simulink model "sm_car_"  (R2026b)
settings: Solver=ode23t  StopTime=100  MaxStep=0.4  AbsTol=1e-3  EnableMultiTasking=on
PreLoadFcn:
  | % Due to usability issue in Repeating Sequence block
  | warning('off','Simulink:Masking:Invalid');
  | 
  | % Eliminate unnecessary warnings in inactive variants
  | % Warnings generated only if you click through inactive variant
  | warning('off','MATLAB:nonExistentField');
  | warning('off','Simulink:Parameters:BlkParamUndefined');
PostLoadFcn:
  | set_param([bdroot '/Vehicle'],'popup_trailer','Off')
  | warning('off','sm:sli:setup:compile:LocalSolverNotSupported')
  | %sm_car_config_maneuver(bdroot,'WOT Braking');
  | sm_car_config_vehicle(bdroot,'false');
  | sm_car_config_logging(bdroot);
InitFcn:
  | sm_car_config_camera;
  | Vehicle = sm_car_vehcfg_checkConfig(Vehicle);
  | sm_car_check_tire_model(bdroot);
StartFcn:
  | tic;
StopFcn:
  | Elapsed_Sim_Time = toc;
  | % disp(['Elapsed Sim Time = ' num2str(Elapsed_Sim_Time)]);
undefined symbols (not defined in the file or in its folder): acc_theta, accel_ramp_rate, Axle1D, AxleIn, Camera, Control, Driver, Init, Maneuver, Pedal, Scene, ShaftL1, ShaftL2, ShaftR1, ShaftR2, Visual, X, xy_data_car_side, Y, Z
libraries: sm_lib x290, fl_lib x171, nesl_utility x144, simulink x60, simulink_extras x14, sdl_lib x14, SimscapeFluids_lib x7, Damper_Element x4, Tire_1x2x x4, ee_lib x3, Scene_Utilities x3, sharedTrackingLibrary x2
(part 20 of 22)

== system sm_car_/Vehicle/Vehicle/Chassis/Spring/Decoupled/Spring A1 Roll/Linear ==
  note: Sensing
  Ctrl : Inport
  Displacement Spring : fl_lib/Mechanical/Mechanical Sensors/Ideal Translational Motion Sensor  reference=foundation.enum.MeasurementReference.difference  acceleration_port=false  velocity_port=true  position_port=true  offset=spr_len0 m
  Force Spring : fl_lib/Mechanical/Mechanical Sensors/Ideal Force Sensor
  PS Term Motion v : fl_lib/Physical Signals/Sinks/PS Terminator
  PS-Simulink Converter : nesl_utility/PS-Simulink Converter  PhysicalDomain=network_engine_domain  SubClassName=ps_output  LeftPortType=input  RightPortType=output  PseudoPeriodic=off  Frequencies=[]  VectorFormat=1-D array  Unit=m  AffineConversion=off
  PS-Simulink Converter1 : nesl_utility/PS-Simulink Converter  PhysicalDomain=network_engine_domain  SubClassName=ps_output  LeftPortType=input  RightPortType=output  PseudoPeriodic=off  Frequencies=[]  VectorFormat=1-D array  Unit=N  AffineConversion=off
  Spring : fl_lib/Mechanical/Translational Elements/Translational Spring  spr_rate=spr_k N/m  v_specify=off  v_priority=None  v=0 m/s  v_nominal_specify=off  v_nominal_value=1  v_nominal_unit=m/s  f_specify=off  f_priority=None  f=0 N  f_nominal_specify=off  f_nominal_value=1  f_nominal_unit=N  x_specify=on  x_priority=High  x=-spr_def0 m  x_nominal_specify=off  x_nominal_value=1  x_nominal_unit=m
  Terminator : Terminator
  R : PMIOPort  Side=Left
  C : PMIOPort  Port=2  Side=Right
  Out Bus Element : Outport  VectorParamsAs1DForOutWhenUnconnected=off  PortName=meas  Element=xSpring
  Out Bus Element1 : Outport  VectorParamsAs1DForOutWhenUnconnected=off  PortName=meas  Element=FSpring
  wires:
  PS-Simulink Converter1/1 -> Out Bus Element1/1
  Ctrl/1 -> Terminator/1
  PS-Simulink Converter/1 -> Out Bus Element/1
  connections:
  Spring/LConn1 -- R/RConn1 -- Displacement Spring/LConn1
  Spring/RConn1 -- Force Spring/RConn1 -- Displacement Spring/RConn1
  Force Spring/LConn1 -- C/RConn1
  PS-Simulink Converter1/LConn1 -- Force Spring/RConn2
  Displacement Spring/RConn2 -- PS Term Motion v/LConn1
  Displacement Spring/RConn3 -- PS-Simulink Converter/LConn1

== system sm_car_/Vehicle/Vehicle/Chassis/Spring/Decoupled/Spring A1 Roll/No Spring ==
  note: Sensor inserted simply to ensure
      | all blocks are connected to a network
  Ctrl : Inport
  Constant : Constant  Value=0
  Constant1 : Constant  Value=0
  Ideal Translational Motion Sensor : fl_lib/Mechanical/Mechanical Sensors/Ideal Translational Motion Sensor  reference=foundation.enum.MeasurementReference.difference  acceleration_port=false  velocity_port=true  position_port=true  offset=0 m
  PS-Simulink Converter : nesl_utility/PS-Simulink Converter  PhysicalDomain=network_engine_domain  SubClassName=ps_output  LeftPortType=input  RightPortType=output  PseudoPeriodic=off  Frequencies=[]  VectorFormat=1-D array  Unit=1  AffineConversion=off
  PS-Simulink Converter1 : nesl_utility/PS-Simulink Converter  PhysicalDomain=network_engine_domain  SubClassName=ps_output  LeftPortType=input  RightPortType=output  PseudoPeriodic=off  Frequencies=[]  VectorFormat=1-D array  Unit=1  AffineConversion=off
  Terminator : Terminator
  Terminator1 : Terminator
  Terminator2 : Terminator
  R : PMIOPort  Side=Left
  C : PMIOPort  Port=2  Side=Right
  Out Bus Element : Outport  VectorParamsAs1DForOutWhenUnconnected=off  PortName=meas  Element=xSpring
  Out Bus Element1 : Outport  VectorParamsAs1DForOutWhenUnconnected=off  PortName=meas  Element=FSpring
  wires:
  PS-Simulink Converter/1 -> Terminator1/1
  PS-Simulink Converter1/1 -> Terminator2/1
  Constant1/1 -> Out Bus Element/1
  Ctrl/1 -> Terminator/1
  Constant/1 -> Out Bus Element1/1
  connections:
  Ideal Translational Motion Sensor/RConn2 -- PS-Simulink Converter/LConn1
  PS-Simulink Converter1/LConn1 -- Ideal Translational Motion Sensor/RConn3
  C/RConn1 -- Ideal Translational Motion Sensor/RConn1
  R/RConn1 -- Ideal Translational Motion Sensor/LConn1

== system sm_car_/Vehicle/Vehicle/Chassis/Spring/Decoupled/Spring A1 Roll/Nonlinear ==
  note: Sensing
  Ctrl : Inport
  Displacement Spring : fl_lib/Mechanical/Mechanical Sensors/Ideal Translational Motion Sensor  reference=foundation.enum.MeasurementReference.difference  acceleration_port=false  velocity_port=true  position_port=true  offset=spr_len0 m
  Force Spring : fl_lib/Mechanical/Mechanical Sensors/Ideal Force Sensor
  PS Term Motion v : fl_lib/Physical Signals/Sinks/PS Terminator
  PS-Simulink Converter : nesl_utility/PS-Simulink Converter  PhysicalDomain=network_engine_domain  SubClassName=ps_output  LeftPortType=input  RightPortType=output  PseudoPeriodic=off  Frequencies=[]  VectorFormat=1-D array  Unit=m  AffineConversion=off
  PS-Simulink Converter1 : nesl_utility/PS-Simulink Converter  PhysicalDomain=network_engine_domain  SubClassName=ps_output  LeftPortType=input  RightPortType=output  PseudoPeriodic=off  Frequencies=[]  VectorFormat=1-D array  Unit=N  AffineConversion=off
  Spring : sdl_lib/Couplings & Drives/Springs & Dampers/Nonlinear Translational Spring  parameterization=2  symmetry=1  coefficient_vector=[100, 0, 10, 0, 1] N/m  tension_coefficient_vector=[100, 0, 10, 0, 1] N/m  compression_coefficient_vector=[1000, -10, 100, 0, 0] N/m  deformation_vector=deformation_vector m  force_vector=force_vector N  interp_method=simscape.enum.interpolation.linear  extrap_method=simscape.enum.extrapolation.linear  x_specify=on  x_priority=High  x=-spr_def0 m  x_nominal_specify=off  x_nominal_value=1  x_nominal_unit=m
  Terminator : Terminator
  R : PMIOPort  Side=Left
  C : PMIOPort  Port=2  Side=Right
  Out Bus Element : Outport  VectorParamsAs1DForOutWhenUnconnected=off  PortName=meas  Element=xSpring
  Out Bus Element1 : Outport  VectorParamsAs1DForOutWhenUnconnected=off  PortName=meas  Element=FSpring
  wires:
  PS-Simulink Converter/1 -> Out Bus Element/1
  Ctrl/1 -> Terminator/1
  PS-Simulink Converter1/1 -> Out Bus Element1/1
  connections:
  Displacement Spring/RConn3 -- PS-Simulink Converter/LConn1
  Displacement Spring/RConn2 -- PS Term Motion v/LConn1
  PS-Simulink Converter1/LConn1 -- Force Spring/RConn2
  Force Spring/LConn1 -- C/RConn1
  Displacement Spring/RConn1 -- Force Spring/RConn1 -- Spring/RConn1
  Displacement Spring/LConn1 -- Spring/LConn1 -- R/RConn1

== system sm_car_/Vehicle/Vehicle/Chassis/Spring/Decoupled/Spring A2 Heave/Linear ==
  note: Sensing
  Ctrl : Inport
  Displacement Spring : fl_lib/Mechanical/Mechanical Sensors/Ideal Translational Motion Sensor  reference=foundation.enum.MeasurementReference.difference  acceleration_port=false  velocity_port=true  position_port=true  offset=spr_len0 m
  Force Spring : fl_lib/Mechanical/Mechanical Sensors/Ideal Force Sensor
  PS Term Motion v : fl_lib/Physical Signals/Sinks/PS Terminator
  PS-Simulink Converter : nesl_utility/PS-Simulink Converter  PhysicalDomain=network_engine_domain  SubClassName=ps_output  LeftPortType=input  RightPortType=output  PseudoPeriodic=off  Frequencies=[]  VectorFormat=1-D array  Unit=m  AffineConversion=off
  PS-Simulink Converter1 : nesl_utility/PS-Simulink Converter  PhysicalDomain=network_engine_domain  SubClassName=ps_output  LeftPortType=input  RightPortType=output  PseudoPeriodic=off  Frequencies=[]  VectorFormat=1-D array  Unit=N  AffineConversion=off
  Spring : fl_lib/Mechanical/Translational Elements/Translational Spring  spr_rate=spr_k N/m  v_specify=off  v_priority=None  v=0 m/s  v_nominal_specify=off  v_nominal_value=1  v_nominal_unit=m/s  f_specify=off  f_priority=None  f=0 N  f_nominal_specify=off  f_nominal_value=1  f_nominal_unit=N  x_specify=on  x_priority=High  x=-spr_def0 m  x_nominal_specify=off  x_nominal_value=1  x_nominal_unit=m
  Terminator : Terminator
  R : PMIOPort  Side=Left
  C : PMIOPort  Port=2  Side=Right
  Out Bus Element : Outport  VectorParamsAs1DForOutWhenUnconnected=off  PortName=meas  Element=xSpring
  Out Bus Element1 : Outport  VectorParamsAs1DForOutWhenUnconnected=off  PortName=meas  Element=FSpring
  wires:
  PS-Simulink Converter1/1 -> Out Bus Element1/1
  Ctrl/1 -> Terminator/1
  PS-Simulink Converter/1 -> Out Bus Element/1
  connections:
  Spring/LConn1 -- R/RConn1 -- Displacement Spring/LConn1
  Spring/RConn1 -- Force Spring/RConn1 -- Displacement Spring/RConn1
  Force Spring/LConn1 -- C/RConn1
  PS-Simulink Converter1/LConn1 -- Force Spring/RConn2
  Displacement Spring/RConn2 -- PS Term Motion v/LConn1
  Displacement Spring/RConn3 -- PS-Simulink Converter/LConn1

== system sm_car_/Vehicle/Vehicle/Chassis/Spring/Decoupled/Spring A2 Heave/No Spring ==
  note: Sensor inserted simply to ensure
      | all blocks are connected to a network
  Ctrl : Inport
  Constant : Constant  Value=0
  Constant1 : Constant  Value=0
  Ideal Translational Motion Sensor : fl_lib/Mechanical/Mechanical Sensors/Ideal Translational Motion Sensor  reference=foundation.enum.MeasurementReference.difference  acceleration_port=false  velocity_port=true  position_port=true  offset=0 m
  PS-Simulink Converter : nesl_utility/PS-Simulink Converter  PhysicalDomain=network_engine_domain  SubClassName=ps_output  LeftPortType=input  RightPortType=output  PseudoPeriodic=off  Frequencies=[]  VectorFormat=1-D array  Unit=1  AffineConversion=off
  PS-Simulink Converter1 : nesl_utility/PS-Simulink Converter  PhysicalDomain=network_engine_domain  SubClassName=ps_output  LeftPortType=input  RightPortType=output  PseudoPeriodic=off  Frequencies=[]  VectorFormat=1-D array  Unit=1  AffineConversion=off
  Terminator : Terminator
  Terminator1 : Terminator
  Terminator2 : Terminator
  R : PMIOPort  Side=Left
  C : PMIOPort  Port=2  Side=Right
  Out Bus Element : Outport  VectorParamsAs1DForOutWhenUnconnected=off  PortName=meas  Element=xSpring
  Out Bus Element1 : Outport  VectorParamsAs1DForOutWhenUnconnected=off  PortName=meas  Element=FSpring
  wires:
  PS-Simulink Converter/1 -> Terminator1/1
  PS-Simulink Converter1/1 -> Terminator2/1
  Constant1/1 -> Out Bus Element/1
  Ctrl/1 -> Terminator/1
  Constant/1 -> Out Bus Element1/1
  connections:
  Ideal Translational Motion Sensor/RConn2 -- PS-Simulink Converter/LConn1
  PS-Simulink Converter1/LConn1 -- Ideal Translational Motion Sensor/RConn3
  C/RConn1 -- Ideal Translational Motion Sensor/RConn1
  R/RConn1 -- Ideal Translational Motion Sensor/LConn1

== system sm_car_/Vehicle/Vehicle/Chassis/Spring/Decoupled/Spring A2 Heave/Nonlinear ==
  note: Sensing
  Ctrl : Inport
  Displacement Spring : fl_lib/Mechanical/Mechanical Sensors/Ideal Translational Motion Sensor  reference=foundation.enum.MeasurementReference.difference  acceleration_port=false  velocity_port=true  position_port=true  offset=spr_len0 m
  Force Spring : fl_lib/Mechanical/Mechanical Sensors/Ideal Force Sensor
  PS Term Motion v : fl_lib/Physical Signals/Sinks/PS Terminator
  PS-Simulink Converter : nesl_utility/PS-Simulink Converter  PhysicalDomain=network_engine_domain  SubClassName=ps_output  LeftPortType=input  RightPortType=output  PseudoPeriodic=off  Frequencies=[]  VectorFormat=1-D array  Unit=m  AffineConversion=off
  PS-Simulink Converter1 : nesl_utility/PS-Simulink Converter  PhysicalDomain=network_engine_domain  SubClassName=ps_output  LeftPortType=input  RightPortType=output  PseudoPeriodic=off  Frequencies=[]  VectorFormat=1-D array  Unit=N  AffineConversion=off
  Spring : sdl_lib/Couplings & Drives/Springs & Dampers/Nonlinear Translational Spring  parameterization=2  symmetry=1  coefficient_vector=[100, 0, 10, 0, 1] N/m  tension_coefficient_vector=[100, 0, 10, 0, 1] N/m  compression_coefficient_vector=[1000, -10, 100, 0, 0] N/m  deformation_vector=deformation_vector m  force_vector=force_vector N  interp_method=simscape.enum.interpolation.linear  extrap_method=simscape.enum.extrapolation.linear  x_specify=on  x_priority=High  x=-spr_def0 m  x_nominal_specify=off  x_nominal_value=1  x_nominal_unit=m
  Terminator : Terminator
  R : PMIOPort  Side=Left
  C : PMIOPort  Port=2  Side=Right
  Out Bus Element : Outport  VectorParamsAs1DForOutWhenUnconnected=off  PortName=meas  Element=xSpring
  Out Bus Element1 : Outport  VectorParamsAs1DForOutWhenUnconnected=off  PortName=meas  Element=FSpring
  wires:
  PS-Simulink Converter/1 -> Out Bus Element/1
  Ctrl/1 -> Terminator/1
  PS-Simulink Converter1/1 -> Out Bus Element1/1
  connections:
  Displacement Spring/RConn3 -- PS-Simulink Converter/LConn1
  Displacement Spring/RConn2 -- PS Term Motion v/LConn1
  PS-Simulink Converter1/LConn1 -- Force Spring/RConn2
  Force Spring/LConn1 -- C/RConn1
  Displacement Spring/RConn1 -- Force Spring/RConn1 -- Spring/RConn1
  Displacement Spring/LConn1 -- Spring/LConn1 -- R/RConn1

== system sm_car_/Vehicle/Vehicle/Chassis/Spring/Decoupled/Spring A2 Roll/Linear ==
  note: Sensing
  Ctrl : Inport
  Displacement Spring : fl_lib/Mechanical/Mechanical Sensors/Ideal Translational Motion Sensor  reference=foundation.enum.MeasurementReference.difference  acceleration_port=false  velocity_port=true  position_port=true  offset=spr_len0 m
  Force Spring : fl_lib/Mechanical/Mechanical Sensors/Ideal Force Sensor
  PS Term Motion v : fl_lib/Physical Signals/Sinks/PS Terminator
  PS-Simulink Converter : nesl_utility/PS-Simulink Converter  PhysicalDomain=network_engine_domain  SubClassName=ps_output  LeftPortType=input  RightPortType=output  PseudoPeriodic=off  Frequencies=[]  VectorFormat=1-D array  Unit=m  AffineConversion=off
  PS-Simulink Converter1 : nesl_utility/PS-Simulink Converter  PhysicalDomain=network_engine_domain  SubClassName=ps_output  LeftPortType=input  RightPortType=output  PseudoPeriodic=off  Frequencies=[]  VectorFormat=1-D array  Unit=N  AffineConversion=off
  Spring : fl_lib/Mechanical/Translational Elements/Translational Spring  spr_rate=spr_k N/m  v_specify=off  v_priority=None  v=0 m/s  v_nominal_specify=off  v_nominal_value=1  v_nominal_unit=m/s  f_specify=off  f_priority=None  f=0 N  f_nominal_specify=off  f_nominal_value=1  f_nominal_unit=N  x_specify=on  x_priority=High  x=-spr_def0 m  x_nominal_specify=off  x_nominal_value=1  x_nominal_unit=m
  Terminator : Terminator
  R : PMIOPort  Side=Left
  C : PMIOPort  Port=2  Side=Right
  Out Bus Element : Outport  VectorParamsAs1DForOutWhenUnconnected=off  PortName=meas  Element=xSpring
  Out Bus Element1 : Outport  VectorParamsAs1DForOutWhenUnconnected=off  PortName=meas  Element=FSpring
  wires:
  PS-Simulink Converter1/1 -> Out Bus Element1/1
  Ctrl/1 -> Terminator/1
  PS-Simulink Converter/1 -> Out Bus Element/1
  connections:
  Spring/LConn1 -- R/RConn1 -- Displacement Spring/LConn1
  Spring/RConn1 -- Force Spring/RConn1 -- Displacement Spring/RConn1
  Force Spring/LConn1 -- C/RConn1
  PS-Simulink Converter1/LConn1 -- Force Spring/RConn2
  Displacement Spring/RConn2 -- PS Term Motion v/LConn1
  Displacement Spring/RConn3 -- PS-Simulink Converter/LConn1

== system sm_car_/Vehicle/Vehicle/Chassis/Spring/Decoupled/Spring A2 Roll/No Spring ==
  note: Sensor inserted simply to ensure
      | all blocks are connected to a network
  Ctrl : Inport
  Constant : Constant  Value=0
  Constant1 : Constant  Value=0
  Ideal Translational Motion Sensor : fl_lib/Mechanical/Mechanical Sensors/Ideal Translational Motion Sensor  reference=foundation.enum.MeasurementReference.difference  acceleration_port=false  velocity_port=true  position_port=true  offset=0 m
  PS-Simulink Converter : nesl_utility/PS-Simulink Converter  PhysicalDomain=network_engine_domain  SubClassName=ps_output  LeftPortType=input  RightPortType=output  PseudoPeriodic=off  Frequencies=[]  VectorFormat=1-D array  Unit=1  AffineConversion=off
  PS-Simulink Converter1 : nesl_utility/PS-Simulink Converter  PhysicalDomain=network_engine_domain  SubClassName=ps_output  LeftPortType=input  RightPortType=output  PseudoPeriodic=off  Frequencies=[]  VectorFormat=1-D array  Unit=1  AffineConversion=off
  Terminator : Terminator
  Terminator1 : Terminator
  Terminator2 : Terminator
  R : PMIOPort  Side=Left
  C : PMIOPort  Port=2  Side=Right
  Out Bus Element : Outport  VectorParamsAs1DForOutWhenUnconnected=off  PortName=meas  Element=xSpring
  Out Bus Element1 : Outport  VectorParamsAs1DForOutWhenUnconnected=off  PortName=meas  Element=FSpring
  wires:
  PS-Simulink Converter/1 -> Terminator1/1
  PS-Simulink Converter1/1 -> Terminator2/1
  Constant1/1 -> Out Bus Element/1
  Ctrl/1 -> Terminator/1
  Constant/1 -> Out Bus Element1/1
  connections:
  Ideal Translational Motion Sensor/RConn2 -- PS-Simulink Converter/LConn1
  PS-Simulink Converter1/LConn1 -- Ideal Translational Motion Sensor/RConn3
  C/RConn1 -- Ideal Translational Motion Sensor/RConn1
  R/RConn1 -- Ideal Translational Motion Sensor/LConn1

== system sm_car_/Vehicle/Vehicle/Chassis/Spring/Decoupled/Spring A2 Roll/Nonlinear ==
  note: Sensing
  Ctrl : Inport
  Displacement Spring : fl_lib/Mechanical/Mechanical Sensors/Ideal Translational Motion Sensor  reference=foundation.enum.MeasurementReference.difference  acceleration_port=false  velocity_port=true  position_port=true  offset=spr_len0 m
  Force Spring : fl_lib/Mechanical/Mechanical Sensors/Ideal Force Sensor
  PS Term Motion v : fl_lib/Physical Signals/Sinks/PS Terminator
  PS-Simulink Converter : nesl_utility/PS-Simulink Converter  PhysicalDomain=network_engine_domain  SubClassName=ps_output  LeftPortType=input  RightPortType=output  PseudoPeriodic=off  Frequencies=[]  VectorFormat=1-D array  Unit=m  AffineConversion=off
  PS-Simulink Converter1 : nesl_utility/PS-Simulink Converter  PhysicalDomain=network_engine_domain  SubClassName=ps_output  LeftPortType=input  RightPortType=output  PseudoPeriodic=off  Frequencies=[]  VectorFormat=1-D array  Unit=N  AffineConversion=off
  Spring : sdl_lib/Couplings & Drives/Springs & Dampers/Nonlinear Translational Spring  parameterization=2  symmetry=1  coefficient_vector=[100, 0, 10, 0, 1] N/m  tension_coefficient_vector=[100, 0, 10, 0, 1] N/m  compression_coefficient_vector=[1000, -10, 100, 0, 0] N/m  deformation_vector=deformation_vector m  force_vector=force_vector N  interp_method=simscape.enum.interpolation.linear  extrap_method=simscape.enum.extrapolation.linear  x_specify=on  x_priority=High  x=-spr_def0 m  x_nominal_specify=off  x_nominal_value=1  x_nominal_unit=m
  Terminator : Terminator
  R : PMIOPort  Side=Left
  C : PMIOPort  Port=2  Side=Right
  Out Bus Element : Outport  VectorParamsAs1DForOutWhenUnconnected=off  PortName=meas  Element=xSpring
  Out Bus Element1 : Outport  VectorParamsAs1DForOutWhenUnconnected=off  PortName=meas  Element=FSpring
  wires:
  PS-Simulink Converter/1 -> Out Bus Element/1
  Ctrl/1 -> Terminator/1
  PS-Simulink Converter1/1 -> Out Bus Element1/1
  connections:
  Displacement Spring/RConn3 -- PS-Simulink Converter/LConn1
  Displacement Spring/RConn2 -- PS Term Motion v/LConn1
  PS-Simulink Converter1/LConn1 -- Force Spring/RConn2
  Force Spring/LConn1 -- C/RConn1
  Displacement Spring/RConn1 -- Force Spring/RConn1 -- Spring/RConn1
  Displacement Spring/LConn1 -- Spring/LConn1 -- R/RConn1

== system sm_car_/Vehicle/Vehicle/Chassis/Spring/Independent/Spring L1/Linear ==
  note: Sensing
  Ctrl : Inport
  Displacement Spring : fl_lib/Mechanical/Mechanical Sensors/Ideal Translational Motion Sensor  reference=foundation.enum.MeasurementReference.difference  acceleration_port=false  velocity_port=true  position_port=true  offset=spr_len0 m
  Force Spring : fl_lib/Mechanical/Mechanical Sensors/Ideal Force Sensor
  Initial Length : Constant  Value=spr_len0
  PS Term Motion v : fl_lib/Physical Signals/Sinks/PS Terminator
  PS-Simulink Converter : nesl_utility/PS-Simulink Converter  PhysicalDomain=network_engine_domain  SubClassName=ps_output  LeftPortType=input  RightPortType=output  PseudoPeriodic=off  Frequencies=[]  VectorFormat=1-D array  Unit=m  AffineConversion=off
  PS-Simulink Converter1 : nesl_utility/PS-Simulink Converter  PhysicalDomain=network_engine_domain  SubClassName=ps_output  LeftPortType=input  RightPortType=output  PseudoPeriodic=off  Frequencies=[]  VectorFormat=1-D array  Unit=N  AffineConversion=off
  Spring : fl_lib/Mechanical/Translational Elements/Translational Spring  spr_rate=spr_k N/m  v_specify=off  v_priority=None  v=0 m/s  v_nominal_specify=off  v_nominal_value=1  v_nominal_unit=m/s  f_specify=off  f_priority=None  f=0 N  f_nominal_specify=off  f_nominal_value=1  f_nominal_unit=N  x_specify=on  x_priority=High  x=-spr_def0 m  x_nominal_specify=off  x_nominal_value=1  x_nominal_unit=m
  Subtract : Sum  Inputs=-+
  Terminator : Terminator
  R : PMIOPort  Side=Left
  C : PMIOPort  Port=2  Side=Right
  Out Bus Element : Outport  VectorParamsAs1DForOutWhenUnconnected=off  PortName=meas  Element=xSpring
  Out Bus Element1 : Outport  VectorParamsAs1DForOutWhenUnconnected=off  PortName=meas  Element=FSpring
  Out Bus Element2 : Outport  VectorParamsAs1DForOutWhenUnconnected=off  PortName=meas  Element=DeltaxSpring
  wires:
  PS-Simulink Converter/1 -> Out Bus Element/1, Subtract/2
  Ctrl/1 -> Terminator/1
  PS-Simulink Converter1/1 -> Out Bus Element1/1
  Initial Length/1 -> Subtract/1
  Subtract/1 -> Out Bus Element2/1
  connections:
  Displacement Spring/RConn3 -- PS-Simulink Converter/LConn1
  Displacement Spring/RConn2 -- PS Term Motion v/LConn1
  PS-Simulink Converter1/LConn1 -- Force Spring/RConn2
  Force Spring/LConn1 -- C/RConn1
  Displacement Spring/RConn1 -- Force Spring/RConn1 -- Spring/RConn1
  Displacement Spring/LConn1 -- R/RConn1 -- Spring/LConn1

== system sm_car_/Vehicle/Vehicle/Chassis/Spring/Independent/Spring L2/Linear ==
  note: Sensing
  Ctrl : Inport
  Displacement Spring : fl_lib/Mechanical/Mechanical Sensors/Ideal Translational Motion Sensor  reference=foundation.enum.MeasurementReference.difference  acceleration_port=false  velocity_port=true  position_port=true  offset=spr_len0 m
  Force Spring : fl_lib/Mechanical/Mechanical Sensors/Ideal Force Sensor
  Initial Length : Constant  Value=spr_len0
  PS Term Motion v : fl_lib/Physical Signals/Sinks/PS Terminator
  PS-Simulink Converter : nesl_utility/PS-Simulink Converter  PhysicalDomain=network_engine_domain  SubClassName=ps_output  LeftPortType=input  RightPortType=output  PseudoPeriodic=off  Frequencies=[]  VectorFormat=1-D array  Unit=m  AffineConversion=off
  PS-Simulink Converter1 : nesl_utility/PS-Simulink Converter  PhysicalDomain=network_engine_domain  SubClassName=ps_output  LeftPortType=input  RightPortType=output  PseudoPeriodic=off  Frequencies=[]  VectorFormat=1-D array  Unit=N  AffineConversion=off
  Spring : fl_lib/Mechanical/Translational Elements/Translational Spring  spr_rate=spr_k N/m  v_specify=off  v_priority=None  v=0 m/s  v_nominal_specify=off  v_nominal_value=1  v_nominal_unit=m/s  f_specify=off  f_priority=None  f=0 N  f_nominal_specify=off  f_nominal_value=1  f_nominal_unit=N  x_specify=on  x_priority=High  x=-spr_def0 m  x_nominal_specify=off  x_nominal_value=1  x_nominal_unit=m
  Subtract : Sum  Inputs=-+
  Terminator : Terminator
  R : PMIOPort  Side=Left
  C : PMIOPort  Port=2  Side=Right
  Out Bus Element : Outport  VectorParamsAs1DForOutWhenUnconnected=off  PortName=meas  Element=xSpring
  Out Bus Element1 : Outport  VectorParamsAs1DForOutWhenUnconnected=off  PortName=meas  Element=FSpring
  Out Bus Element2 : Outport  VectorParamsAs1DForOutWhenUnconnected=off  PortName=meas  Element=DeltaxSpring
  wires:
  PS-Simulink Converter1/1 -> Out Bus Element1/1
  Ctrl/1 -> Terminator/1
  Subtract/1 -> Out Bus Element2/1
  PS-Simulink Converter/1 -> Subtract/2, Out Bus Element/1
  Initial Length/1 -> Subtract/1
  connections:
  Spring/LConn1 -- R/RConn1 -- Displacement Spring/LConn1
  Spring/RConn1 -- Force Spring/RConn1 -- Displacement Spring/RConn1
  Force Spring/LConn1 -- C/RConn1
  PS-Simulink Converter1/LConn1 -- Force Spring/RConn2
  Displacement Spring/RConn2 -- PS Term Motion v/LConn1
  Displacement Spring/RConn3 -- PS-Simulink Converter/LConn1

== system sm_car_/Vehicle/Vehicle/Chassis/Spring/Independent/Spring R1/Linear ==
  note: Sensing
  Ctrl : Inport
  Displacement Spring : fl_lib/Mechanical/Mechanical Sensors/Ideal Translational Motion Sensor  reference=foundation.enum.MeasurementReference.difference  acceleration_port=false  velocity_port=true  position_port=true  offset=spr_len0 m
  Force Spring : fl_lib/Mechanical/Mechanical Sensors/Ideal Force Sensor
  Initial Length : Constant  Value=spr_len0
  PS Term Motion v : fl_lib/Physical Signals/Sinks/PS Terminator
  PS-Simulink Converter : nesl_utility/PS-Simulink Converter  PhysicalDomain=network_engine_domain  SubClassName=ps_output  LeftPortType=input  RightPortType=output  PseudoPeriodic=off  Frequencies=[]  VectorFormat=1-D array  Unit=m  AffineConversion=off
  PS-Simulink Converter1 : nesl_utility/PS-Simulink Converter  PhysicalDomain=network_engine_domain  SubClassName=ps_output  LeftPortType=input  RightPortType=output  PseudoPeriodic=off  Frequencies=[]  VectorFormat=1-D array  Unit=N  AffineConversion=off
  Spring : fl_lib/Mechanical/Translational Elements/Translational Spring  spr_rate=spr_k N/m  v_specify=off  v_priority=None  v=0 m/s  v_nominal_specify=off  v_nominal_value=1  v_nominal_unit=m/s  f_specify=off  f_priority=None  f=0 N  f_nominal_specify=off  f_nominal_value=1  f_nominal_unit=N  x_specify=on  x_priority=High  x=-spr_def0 m  x_nominal_specify=off  x_nominal_value=1  x_nominal_unit=m
  Subtract : Sum  Inputs=-+
  Terminator : Terminator
  R : PMIOPort  Side=Left
  C : PMIOPort  Port=2  Side=Right
  Out Bus Element : Outport  VectorParamsAs1DForOutWhenUnconnected=off  PortName=meas  Element=xSpring
  Out Bus Element1 : Outport  VectorParamsAs1DForOutWhenUnconnected=off  PortName=meas  Element=FSpring
  Out Bus Element2 : Outport  VectorParamsAs1DForOutWhenUnconnected=off  PortName=meas  Element=DeltaxSpring
  wires:
  PS-Simulink Converter1/1 -> Out Bus Element1/1
  Ctrl/1 -> Terminator/1
  Subtract/1 -> Out Bus Element2/1
  PS-Simulink Converter/1 -> Subtract/2, Out Bus Element/1
  Initial Length/1 -> Subtract/1
  connections:
  Spring/LConn1 -- R/RConn1 -- Displacement Spring/LConn1
  Spring/RConn1 -- Displacement Spring/RConn1 -- Force Spring/RConn1
  Force Spring/LConn1 -- C/RConn1
  PS-Simulink Converter1/LConn1 -- Force Spring/RConn2
  Displacement Spring/RConn2 -- PS Term Motion v/LConn1
  Displacement Spring/RConn3 -- PS-Simulink Converter/LConn1

== system sm_car_/Vehicle/Vehicle/Chassis/Spring/Independent/Spring R2/Linear ==
  note: Sensing
  Ctrl : Inport
  Displacement Spring : fl_lib/Mechanical/Mechanical Sensors/Ideal Translational Motion Sensor  reference=foundation.enum.MeasurementReference.difference  acceleration_port=false  velocity_port=true  position_port=true  offset=spr_len0 m
  Force Spring : fl_lib/Mechanical/Mechanical Sensors/Ideal Force Sensor
  Initial Length : Constant  Value=spr_len0
  PS Term Motion v : fl_lib/Physical Signals/Sinks/PS Terminator
  PS-Simulink Converter : nesl_utility/PS-Simulink Converter  PhysicalDomain=network_engine_domain  SubClassName=ps_output  LeftPortType=input  RightPortType=output  PseudoPeriodic=off  Frequencies=[]  VectorFormat=1-D array  Unit=m  AffineConversion=off
  PS-Simulink Converter1 : nesl_utility/PS-Simulink Converter  PhysicalDomain=network_engine_domain  SubClassName=ps_output  LeftPortType=input  RightPortType=output  PseudoPeriodic=off  Frequencies=[]  VectorFormat=1-D array  Unit=N  AffineConversion=off
  Spring : fl_lib/Mechanical/Translational Elements/Translational Spring  spr_rate=spr_k N/m  v_specify=off  v_priority=None  v=0 m/s  v_nominal_specify=off  v_nominal_value=1  v_nominal_unit=m/s  f_specify=off  f_priority=None  f=0 N  f_nominal_specify=off  f_nominal_value=1  f_nominal_unit=N  x_specify=on  x_priority=High  x=-spr_def0 m  x_nominal_specify=off  x_nominal_value=1  x_nominal_unit=m
  Subtract : Sum  Inputs=-+
  Terminator : Terminator
  R : PMIOPort  Side=Left
  C : PMIOPort  Port=2  Side=Right
  Out Bus Element : Outport  VectorParamsAs1DForOutWhenUnconnected=off  PortName=meas  Element=xSpring
  Out Bus Element1 : Outport  VectorParamsAs1DForOutWhenUnconnected=off  PortName=meas  Element=FSpring
  Out Bus Element2 : Outport  VectorParamsAs1DForOutWhenUnconnected=off  PortName=meas  Element=DeltaxSpring
  wires:
  PS-Simulink Converter1/1 -> Out Bus Element1/1
  Ctrl/1 -> Terminator/1
  Subtract/1 -> Out Bus Element2/1
  PS-Simulink Converter/1 -> Out Bus Element/1, Subtract/2
  Initial Length/1 -> Subtract/1
  connections:
  Spring/LConn1 -- R/RConn1 -- Displacement Spring/LConn1
  Spring/RConn1 -- Force Spring/RConn1 -- Displacement Spring/RConn1
  Force Spring/LConn1 -- C/RConn1
  PS-Simulink Converter1/LConn1 -- Force Spring/RConn2
  Displacement Spring/RConn2 -- PS Term Motion v/LConn1
  Displacement Spring/RConn3 -- PS-Simulink Converter/LConn1

== system sm_car_/Vehicle/Vehicle/Powertrain/Driveline/L2 R2/ShaftL1/Driveshaft Measurements ==
  Bus Creator : BusCreator  Inputs=2
  Zero : Constant  Value=0  OutDataTypeStr=Inherit: Inherit via back propagation
  Zero1 : Constant  Value=0  OutDataTypeStr=Inherit: Inherit via back propagation
  meas : Outport  VectorParamsAs1DForOutWhenUnconnected=off
  wires:
  Zero/1 -> Bus Creator/1  "w"
  Zero1/1 -> Bus Creator/2  "q"
  Bus Creator/1 -> meas/1

== system sm_car_/Vehicle/Vehicle/Powertrain/Driveline/L2 R2/ShaftR1/Driveshaft Measurements ==
  Bus Creator : BusCreator  Inputs=2
  Zero : Constant  Value=0  OutDataTypeStr=Inherit: Inherit via back propagation
  Zero1 : Constant  Value=0  OutDataTypeStr=Inherit: Inherit via back propagation
  meas : Outport  VectorParamsAs1DForOutWhenUnconnected=off
  wires:
  Zero/1 -> Bus Creator/1  "w"
  Zero1/1 -> Bus Creator/2  "q"
  Bus Creator/1 -> meas/1

== system sm_car_/Vehicle/Vehicle/Powertrain/Power/Electric L2 R2/Battery/Sensor VI ==
  Bus Creator : BusCreator  Inputs=2
  Current Sensor : fl_lib/Electrical/Electrical Sensors/Current Sensor
  PS-Simulink Converter2 : nesl_utility/PS-Simulink Converter  PhysicalDomain=network_engine_domain  SubClassName=ps_output  LeftPortType=input  RightPortType=output  PseudoPeriodic=off  Frequencies=[]  VectorFormat=1-D array  Unit=1  AffineConversion=off
  PS-Simulink Converter4 : nesl_utility/PS-Simulink Converter  PhysicalDomain=network_engine_domain  SubClassName=ps_output  LeftPortType=input  RightPortType=output  PseudoPeriodic=off  Frequencies=[]  VectorFormat=1-D array  Unit=1  AffineConversion=off
  Transfer Fcn1 : TransferFcn  Denominator=[.001 1]
  Transfer Fcn5 : TransferFcn  Denominator=[.001 1]
  Voltage Sensor2 : fl_lib/Electrical/Electrical Sensors/Voltage Sensor
  + : PMIOPort  Side=Left
  - : PMIOPort  Port=2  Side=Right
  G : PMIOPort  Port=3  Side=Right
  vi : Outport
  wires:
  Bus Creator/1 -> vi/1
  Transfer Fcn5/1 -> Bus Creator/1  "v"
  Transfer Fcn1/1 -> Bus Creator/2  "i"
  PS-Simulink Converter2/1 -> Transfer Fcn1/1
  PS-Simulink Converter4/1 -> Transfer Fcn5/1
  connections:
  Current Sensor/RConn1 -- PS-Simulink Converter2/LConn1
  Voltage Sensor2/RConn2 -- G/RConn1
  Current Sensor/RConn2 -- -/RConn1
  PS-Simulink Converter4/LConn1 -- Voltage Sensor2/RConn1
  Voltage Sensor2/LConn1 -- Current Sensor/LConn1 -- +/RConn1

== system sm_car_/Vehicle/Vehicle/Powertrain/Power/Electric L2 R2/Motor L2/Sensing Current ==
  Current Sensor : fl_lib/Electrical/Electrical Sensors/Current Sensor
  PS-Simulink Converter1 : nesl_utility/PS-Simulink Converter  PhysicalDomain=network_engine_domain  SubClassName=ps_output  LeftPortType=input  RightPortType=output  PseudoPeriodic=off  Frequencies=[]  VectorFormat=1-D array  Unit=1  AffineConversion=off
  + : PMIOPort  Side=Right
  - : PMIOPort  Port=2  Side=Left
  Out1 : Outport  VectorParamsAs1DForOutWhenUnconnected=off
  wires:
  PS-Simulink Converter1/1 -> Out1/1
  connections:
  +/RConn1 -- Current Sensor/LConn1
  Current Sensor/RConn1 -- PS-Simulink Converter1/LConn1
  Current Sensor/RConn2 -- -/RConn1

== system sm_car_/Vehicle/Vehicle/Powertrain/Power/Electric L2 R2/Motor L2/Sensing Torque ==
  Ideal Torque Sensor : fl_lib/Mechanical/Mechanical Sensors/Ideal Torque Sensor
  PS-Simulink Converter1 : nesl_utility/PS-Simulink Converter  PhysicalDomain=network_engine_domain  SubClassName=ps_output  LeftPortType=input  RightPortType=output  PseudoPeriodic=off  Frequencies=[]  VectorFormat=1-D array  Unit=1  AffineConversion=off
  R : PMIOPort  Side=Left
  C : PMIOPort  Port=2  Side=Right
  T : Outport  VectorParamsAs1DForOutWhenUnconnected=off
  wires:
  PS-Simulink Converter1/1 -> T/1
  connections:
  Ideal Torque Sensor/LConn1 -- R/RConn1
  Ideal Torque Sensor/RConn1 -- C/RConn1
  Ideal Torque Sensor/RConn2 -- PS-Simulink Converter1/LConn1

== system sm_car_/Vehicle/Vehicle/Powertrain/Power/Electric L2 R2/Motor R2/Sensing Current ==
  Current Sensor : fl_lib/Electrical/Electrical Sensors/Current Sensor
  PS-Simulink Converter1 : nesl_utility/PS-Simulink Converter  PhysicalDomain=network_engine_domain  SubClassName=ps_output  LeftPortType=input  RightPortType=output  PseudoPeriodic=off  Frequencies=[]  VectorFormat=1-D array  Unit=1  AffineConversion=off
  + : PMIOPort  Side=Right
  - : PMIOPort  Port=2  Side=Left
  Out1 : Outport  VectorParamsAs1DForOutWhenUnconnected=off
  wires:
  PS-Simulink Converter1/1 -> Out1/1
  connections:
  +/RConn1 -- Current Sensor/LConn1
  Current Sensor/RConn1 -- PS-Simulink Converter1/LConn1
  Current Sensor/RConn2 -- -/RConn1

== system sm_car_/Vehicle/Vehicle/Powertrain/Power/Electric L2 R2/Motor R2/Sensing Torque ==
  Ideal Torque Sensor : fl_lib/Mechanical/Mechanical Sensors/Ideal Torque Sensor
  PS-Simulink Converter1 : nesl_utility/PS-Simulink Converter  PhysicalDomain=network_engine_domain  SubClassName=ps_output  LeftPortType=input  RightPortType=output  PseudoPeriodic=off  Frequencies=[]  VectorFormat=1-D array  Unit=1  AffineConversion=off
  R : PMIOPort  Side=Left
  C : PMIOPort  Port=2  Side=Right
  T : Outport  VectorParamsAs1DForOutWhenUnconnected=off
  wires:
  PS-Simulink Converter1/1 -> T/1
  connections:
  Ideal Torque Sensor/LConn1 -- R/RConn1
  Ideal Torque Sensor/RConn1 -- C/RConn1
  Ideal Torque Sensor/RConn2 -- PS-Simulink Converter1/LConn1
